simulink model "BatterySOCEstimation"  (R2025b)
settings: Solver=VariableStepAuto  StartTime=0.0  StopTime=6*3600  FixedStep=Ts  RelTol=1e-3  EnableMultiTasking=on
PreLoadFcn:
  | BatterySOCEstimationData;
values from neighbouring files (symbols this model uses):
  R = 0.7    [BatterySOCEstimationData.m]    (also in UTFRBatteryParameters.m = 0.5)
  SOC0 = 0.8    [BatterySOCEstimationData.m]    (also in UTFRBatteryParameters.m = 0.95)
  Ts = 1    [BatterySOCEstimationData.m]    (also in UTFRBatteryParameters.m = 0.01)
libraries: fl_lib x8, nesl_utility x5, simulink x3, batteryecm_lib x1, BatteryEstimators x1
CloseFcn:
  | try
  |     close(h1_BatterySOCEstimation)
  | catch
  | end
  | 
  | clear h1_BatterySOCEstimation
  | 
  | clear BatterySOCEstimationSimlog
  | clear BatterySOCEstimationLogsout
  | 
  | clear AH SOC_vec T_vec R0_mat R1_mat tau1_mat
  | clear V0_mat Q R P0 initialSOC SOC0 Ts
  | clear cell_area h_conv thermal_mass
Description:
  | Battery State-of-Charge Estimation
settings Model: Creator=The MathWorks, Inc.  LastModifiedBy=The MathWorks, Inc.
settings SolverCC: AlgebraicLoopSolver=TrustRegion  AutoInsertRateTranBlk=on  MaxZcPerStep=1.0
settings DataIOCC: MaxDataPoints=370000  ReturnWorkspaceOutputs=off  SignalLoggingName=BatterySOCEstimationLogsout
settings OptimizationCC: ReuseModelBlockBuffer=off  LifeSpan=inf
settings DebuggingCC: UnconnectedInputMsg=warning  UnconnectedOutputMsg=warning  UnconnectedLineMsg=warning  SFUnexpectedBacktrackingDiag=warning  SFNoUnconditionalDefaultTransitionDiag=warning  SFExecutionAtInitializationDiag=none  ArithmeticOperatorsInVariantConditions=warning
settings ModelReferenceCC: EnableRefExpFcnMdlSchedulingChecks=on
settings SFSimCC: SimUseLocalCustomCode=off  CustomCodeUndefinedFunction=UseInterfaceOnly
settings RTWCC: RTWUseLocalCustomCode=off  GPUComputeCapability=3.5  DLArmComputeVersion=19.05
settings CodeAppCC: StateflowObjectComments=on
settings GRTTargetCC: TargetLangStandard=C89/C90 (ANSI)
settings ConfigComp: CovMetricSettings=dw  CovSaveCumulativeToWorkspaceVar=on  CovSaveSingleToWorkspaceVar=on  CovExternalEMLEnable=off
settings SimscapeCC: SimscapeLogType=all  SimscapeLogSimulationStatistics=on  SimscapeLogName=BatterySOCEstimationSimlog  SimscapeLogLimitData=off  SimscapeLogDataHistory=370000.0

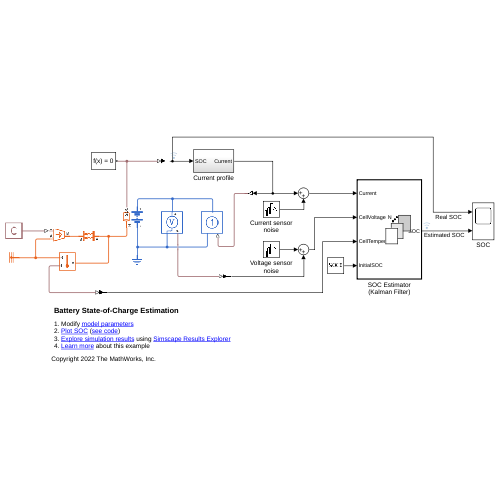
[thumbnail: Simulink's stored preview of the top-level diagram]
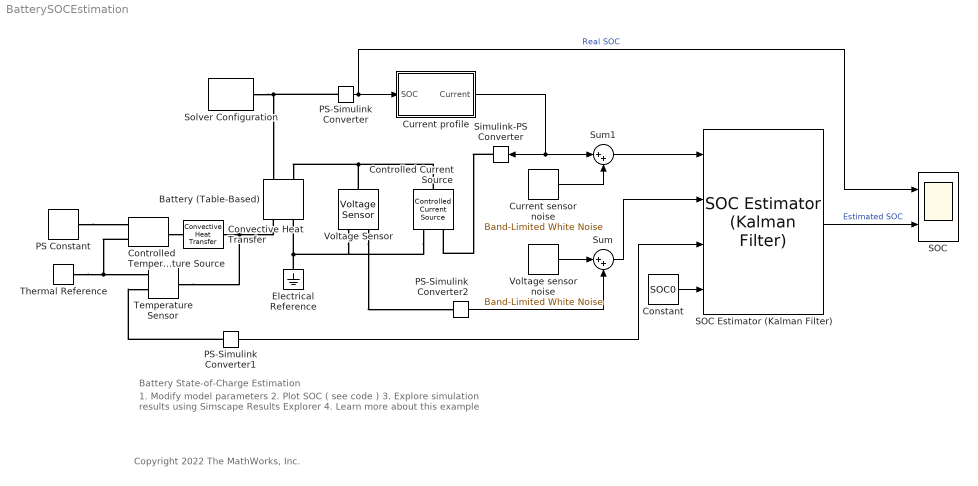
== system BatterySOCEstimation ==
  note: Battery State-of-Charge Estimation
  note: 1. Modify model parameters
      | 2. Plot SOC ( see code )
      | 3. Explore simulation results using Simscape Results Explorer
      | 4. Learn more about this example
  note: Copyright 2022 The MathWorks, Inc.
  Battery (Table-Based) : batteryecm_lib/Battery (Table-Based)  SOC_vec=SOC_vec  T_dependence=simscape.enum.tablebattery.temperature_dependence.yes  prm_dir=simscape.enum.tablebattery.prm_dir.noCurrentDirectionality  T_vec=T_vec K  V0_mat=V0_mat V  V0_vec=[3.5057, 3.566, 3.6337, 3.7127, 3.9259, 4.0777, 4.1928] V  V_range=[0, inf] V  R0_mat=R0_mat Ohm  R0_vec=[.0085, .0085, .0087, .0082, .0083, .0085, .0085] Ohm  R0_dis_mat=[.0117, .0085, .009; .011, .0085, .009; .0114, .0087, .0092; .0107, .0082, .0088; .0107, .0083, .0091; .0113, .0085, .0089; .0116, .0085, .0089] Ohm  R0_dis_vec=[.0085, .0085, .0087, .0082, .0083, .0085, .0085] Ohm  R0_ch_mat=[.0117, .0085, .009; .011, .0085, .009; .0114, .0087, .0092; .0107, .0082, .0088; .0107, .0083, .0091; .0113, .0085, .0089; .0116, .0085, .0089] Ohm  R0_ch_vec=[.0085, .0085, .0087, .0082, .0083, .0085, .0085] Ohm  AH=AH A*hr  prm_leak=simscape.enum.tablebattery.prm_leak.disabled  Rleak_vec=[8000, 7000, 6000] Ohm  Rleak=7e3 Ohm  extrapolation_option=simscape.enum.extrapolation.nearest  SOC_port=simscape.enum.tablebattery.enable.yes  prm_dyn=simscape.enum.tablebattery.prm_dyn.rc1  R1_mat=R1_mat Ohm  R1_vec=[.0029, .0024, .0026, .0016, .0023, .0018, .0017] Ohm  tau1_mat=tau1_mat s  tau1_vec=[36, 45, 105, 29, 77, 33, 39] s  R2_mat=[.0109, .0029, .0013; .0069, .0024, .0012; .0047, .0026, .0013; .0034, .0016, .001; .0033, .0023, .0014; .0033, .0018, .0011; .0028, .0017, .0011] Ohm  R2_vec=[.0029, .0024, .0026, .0016, .0023, .0018, .0017] Ohm  tau2_mat=[20, 36, 39; 31, 45, 39; 109, 105, 61; 36, 29, 26; 59, 77, 67; 40, 33, 29; 25, 39, 33] s  tau2_vec=[36, 45, 105, 29, 77, 33, 39] s  R3_mat=[.0109, .0029, .0013; .0069, .0024, .0012; .0047, .0026, .0013; .0034, .0016, .001; .0033, .0023, .0014; .0033, .0018, .0011; .0028, .0017, .0011] Ohm  R3_vec=[.0029, .0024, .0026, .0016, .0023, .0018, .0017] Ohm  tau3_mat=[20, 36, 39; 31, 45, 39; 109, 105, 61; 36, 29, 26; 59, 77, 67; 40, 33, 29; 25, 39, 33] s  tau3_vec=[36, 45, 105, 29, 77, 33, 39] s  R4_mat=[.0109, .0029, .0013; .0069, .0024, .0012; .0047, .0026, .0013; .0034, .0016, .001; .0033, .0023, .0014; .0033, .0018, .0011; .0028, .0017, .0011] Ohm  R4_vec=[.0029, .0024, .0026, .0016, .0023, .0018, .0017] Ohm  tau4_mat=[20, 36, 39; 31, 45, 39; 109, 105, 61; 36, 29, 26; 59, 77, 67; 40, 33, 29; 25, 39, 33] s  tau4_vec=[36, 45, 105, 29, 77, 33, 39] s  R5_mat=[.0109, .0029, .0013; .0069, .0024, .0012; .0047, .0026, .0013; .0034, .0016, .001; .0033, .0023, .0014; .0033, .0018, .0011; .0028, .0017, .0011] Ohm  R5_vec=[.0029, .0024, .0026, .0016, .0023, .0018, .0017] Ohm  tau5_mat=[20, 36, 39; 31, 45, 39; 109, 105, 61; 36, 29, 26; 59, 77, 67; 40, 33, 29; 25, 39, 33] s  tau5_vec=[36, 45, 105, 29, 77, 33, 39] s  prm_fade=simscape.enum.tablebattery.prm_fade.disabled  N0=10  dV0=0  dR0=500  dAH=0  dRleak=0  dR1=0  dR2=0  dR3=0  dR4=0  dR5=0  N0vec=[100, 200, 300]  Tfadevec=[298.15, 323.15] K  dV0vec=[0, 0, 0]  dR0vec=[0, 0, 0]  dAHvec=[0, 0, 0]  dRleakvec=[0, 0, 0]  dR1vec=[0, 0, 0]  dR2vec=[0, 0, 0]  dR3vec=[0, 0, 0]  dR4vec=[0, 0, 0]  dR5vec=[0, 0, 0]  dV0mat=[0, 0; 0, 0; 0, 0]  dR0mat=[0, 0; 0, 0; 0, 0]  dAHmat=[0, 0; 0, 0; 0, 0]  dRleakmat=[0, 0; 0, 0; 0, 0]  dR1mat=[0, 0; 0, 0; 0, 0]  dR2mat=[0, 0; 0, 0; 0, 0]  dR3mat=[0, 0; 0, 0; 0, 0]  dR4mat=[0, 0; 0, 0; 0, 0]  dR5mat=[0, 0; 0, 0; 0, 0]  prm_age_modeling=simscape.enum.tablebattery.prm_age_modeling.equation  storage_dt_age_vec=[0] d  storage_T_age_vec=[273] K  prm_age_OCV=simscape.enum.tablebattery.prm_age_OCV.OCV  OCV_age=0.9  SOC_age=0.6  prm_age_resistance=simscape.enum.tablebattery.prm_age.disabled  OCV_scaling_age_resistance=2.2134e6  OCV_offset_age_resistance=1.632e6  temp_exp_age_resistance=0.515833569 V  t_exp_age_resistance=0.75  T_age_vec_resistance=[273.15, 298.15, 323.15] K  dt_age_vec_resistance=[90, 180, 270, 360] d  dR0_age_vec=[0, 0, 0]  t_meas_dR0_age=100 d  dR0_age_mat=[0, 0, 0; 0, 0, 0; 0, 0, 0; 0, 0, 0]  prm_age_capacity=simscape.enum.tablebattery.prm_age.disabled  OCV_scaling_age_capacity=1.5097e07  OCV_offset_age_capacity=8.3625e06  temp_exp_age_capacity=0.6011 V  t_exp_age_capacity=0.75  T_age_vec_capacity=[273.15, 298.15, 323.15] K  dt_age_vec_capacity=[90, 180, 270, 360] d  dAH_age_vec=[0, 0, 0]  t_meas_dAH_age=100 d  dAH_age_mat=[0, 0, 0; 0, 0, 0; 0, 0, 0; 0, 0, 0]  thermal_port=simscape.enum.thermaleffects.model  temperature=298.15 K  thermal_mass=thermal_mass J/K  i_specify=off  i_priority=None  i=0 A  i_nominal_specify=off  i_nominal_value=1  i_nominal_unit=A  v_specify=off  v_priority=None  v=0 V  v_nominal_specify=off  v_nominal_value=1  v_nominal_unit=V  stateOfCharge_specify=on  stateOfCharge_priority=High  stateOfCharge=initialSOC  stateOfCharge_nominal_specify=off  stateOfCharge_nominal_value=1  stateOfCharge_nominal_unit=1  num_cycles_specify=off  num_cycles_priority=High  num_cycles=0  num_cycles_nominal_specify=off  num_cycles_nominal_value=1  num_cycles_nominal_unit=1  cell_temperature_specify=off  cell_temperature_priority=High  cell_temperature=293.15 K  cell_temperature_nominal_specify=off  cell_temperature_nominal_value=1  cell_temperature_nominal_unit=K
  Constant : Constant  Value=SOC0
  Controlled Temperature Source : fl_lib/Thermal/Thermal Sources/Controlled Temperature Source
  Controlled Current Source : fl_lib/Electrical/Electrical Sources/Controlled Current Source
  Convective Heat Transfer : fl_lib/Thermal/Thermal Elements/Convective Heat Transfer  thermal_type=foundation.enum.constant_variable.constant  area=cell_area m^2  heat_tr_coeff=h_conv W/(K*m^2)  min_heat_tr_coeff=1e-3 W/(K*m^2)  T_specify=off  T_priority=None  T=0 K  T_nominal_specify=off  T_nominal_value=1  T_nominal_unit=K  Q_specify=off  Q_priority=None  Q=0 W  Q_nominal_specify=off  Q_nominal_value=1  Q_nominal_unit=W
  Current profile : Subsystem
  Current sensor noise : simulink/Sources/Band-Limited White Noise  Cov=1e-2  Ts=1  seed=1234
  Electrical Reference : fl_lib/Electrical/Electrical Elements/Electrical Reference
  PS Constant : fl_lib/Physical Signals/Sources/PS Constant  constant=292.15 K
  PS-Simulink Converter : nesl_utility/PS-Simulink Converter  PhysicalDomain=network_engine_domain  SubClassName=ps_output  LeftPortType=input  RightPortType=output  PseudoPeriodic=off  Frequencies=[]  VectorFormat=inherit  Unit=inherit  AffineConversion=off
  PS-Simulink Converter1 : nesl_utility/PS-Simulink Converter  PhysicalDomain=network_engine_domain  SubClassName=ps_output  LeftPortType=input  RightPortType=output  PseudoPeriodic=off  Frequencies=[]  VectorFormat=inherit  Unit=inherit  AffineConversion=off
  PS-Simulink Converter2 : nesl_utility/PS-Simulink Converter  PhysicalDomain=network_engine_domain  SubClassName=ps_output  LeftPortType=input  RightPortType=output  PseudoPeriodic=off  Frequencies=[]  VectorFormat=inherit  Unit=inherit  AffineConversion=off
  SOC : Scope  NumInputPorts=2
      settings: ActiveDisplayYMinimum=0.20845  ActiveDisplayYMaximum=0.98731  DataLoggingVariableName=ScopeData3
  SOC Estimator (Kalman Filter) : BatteryEstimators/SOC Estimator (Kalman Filter)  CurrentInputPartition=off  filterType=Extended Kalman filter  alpha=1  beta=2  kappa=0  Q=Q  Q_2RC=|  R=R  P0=P0  P0_2RC=[1e-5 0 0; 0 1 0;0 0 1]  Ts=Ts  chargeDynamics=One time-constant dynamics  SOC_vec=SOC_vec  T_vec=T_vec  R0_mat=R0_mat  R1_mat=R1_mat  tau1_mat=tau1_mat  R2_mat=[.0109, .0029, .0013; .0069, .0024, .0012; .0047, .0026, .0013; .0034, .0016, .001; .0033, .0023, .0014; .0033, .0018, .0011; .0028, .0017, .0011]  tau2_mat=[20, 36, 39; 31, 45, 39; 109, 105, 61; 36, 29, 26; 59, 77, 67; 40, 33, 29; 25, 39, 33]  V0_mat=V0_mat  AH=AH  DataType=Inherit: auto
      | [1e-6 0 0;
      | 0 1e-6 0; 0 0 1e-6]
  Simulink-PS Converter : nesl_utility/Simulink-PS Converter  PhysicalDomain=network_engine_domain  SubClassName=ps_input  LeftPortType=input  RightPortType=output  PseudoPeriodic=off  Frequencies=[]  NoiseDistribution=none  NoiseParameters=[]  Unit=1  AffineConversion=off  FilteringAndDerivatives=provide  SimscapeFilterOrder=1  InputFilterTimeConstant=0.001  UdotUserProvided=0
  Solver Configuration : nesl_utility/Solver Configuration  PhysicalDomain=network_engine_domain  SubClassName=solver  LeftPortType=input  RightPortType=generic  Tones=[]  Harmonics=[]  SimulateNoise=off  Profile=off  UseLocalSampling=off  EnableSwitchedLinearOptims=on  FrequencyDomain=off  UseCCode=off  RelTol=0.001  AbsTol=0.001  MinStep=1e-09  ToWorkspace=off  RevertToSquareIcSolve=off  NumHomotopyIterations=100  PhasorMode=off  PhasorModeNumHarmonics=1  ConsistencySolver=NEWTON_XTOL_AFTER_FTOL  IndexReductionMethod=DerivativeReplacement  DoDC=off  ResidualTolerance=1e-09  ConsistencyTolSource=GLOBAL  ConsistencyAbsTol=0.001  ConsistencyRelTol=0.001  ConsistencyTolFactor=0.001  UseLocalSolver=on  LocalSolverChoice=NE_BACKWARD_EULER_ADVANCER  ResolveIndetEquations=on  FunctionEvalNumThread=1  LocalSolverSampleTime=1  DoFixedCost=on  MaxNonlinIter=3  MaxModeIter=2  ComputeImpulses=off  ImpulseIterations=2  LinearAlgebra=auto  LinearAlgebraNumThread=0  EquationFormulation=NE_TIME_EF  DelaysMemoryBudget=1024  AutomaticFiltering=on  FilteringTimeConstant=0.001  PartitionStorageMethod=AS_NEEDED  PartitionMemoryBudget=1024  PartitionMethod=ROBUST  MultibodyUseLocalSolver=off  MultibodyLocalSolverChoice=ODE1  MultibodyLocalSolverSampleTime=0.001
  Sum : Sum  Inputs=|++
  Sum1 : Sum  Inputs=|++
  Temperature Sensor : fl_lib/Thermal/Thermal Sensors/Temperature Sensor  temperature_measure=foundation.enum.MeasurementReference.difference
  Thermal Reference : fl_lib/Thermal/Thermal Elements/Thermal Reference
  Voltage Sensor : fl_lib/Electrical/Electrical Sensors/Voltage Sensor
  Voltage sensor noise : simulink/Sources/Band-Limited White Noise  Cov=1e-2  Ts=1  seed=1234
  wires:
  PS-Simulink Converter2/1 -> Sum/2
  Current sensor noise/1 -> Sum1/2
  Sum1/1 -> SOC Estimator (Kalman Filter)/1
  Sum/1 -> SOC Estimator (Kalman Filter)/2
  PS-Simulink Converter1/1 -> SOC Estimator (Kalman Filter)/3
  Constant/1 -> SOC Estimator (Kalman Filter)/4
  SOC Estimator (Kalman Filter)/1 -> SOC/2  "Estimated SOC"
  PS-Simulink Converter/1 -> SOC/1, Current profile/1(SOC)  "Real SOC"
  Voltage sensor noise/1 -> Sum/1
  Current profile/1(Current) -> Sum1/1, Simulink-PS Converter/1
  connections:
  PS-Simulink Converter/LConn1 -- Solver Configuration/RConn1 -- Battery (Table-Based)/LConn2
  Convective Heat Transfer/LConn1 -- Temperature Sensor/LConn1 -- Battery (Table-Based)/RConn2
  Controlled Temperature Source/LConn1 -- Convective Heat Transfer/RConn1
  Thermal Reference/LConn1 -- Controlled Temperature Source/RConn2 -- Temperature Sensor/RConn1
  PS-Simulink Converter1/LConn1 -- Temperature Sensor/RConn2
  Electrical Reference/LConn1 -- Voltage Sensor/RConn2 -- Controlled Current Source/RConn2 -- Battery (Table-Based)/RConn1
  Voltage Sensor/LConn1 -- Controlled Current Source/LConn1 -- Battery (Table-Based)/LConn1
  Simulink-PS Converter/RConn1 -- Controlled Current Source/RConn1
  Voltage Sensor/RConn1 -- PS-Simulink Converter2/LConn1
  PS Constant/RConn1 -- Controlled Temperature Source/RConn1

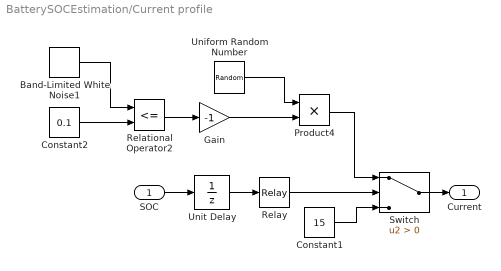
== system BatterySOCEstimation/Current profile ==
  SOC : Inport
  Band-Limited White Noise1 : simulink/Sources/Band-Limited White Noise  Cov=1  Ts=50  seed=[23341]
  Constant1 : Constant  Value=15
  Constant2 : Constant  Value=0.1
  Gain : Gain  Gain=-1
  Product4 : Product
  Relational Operator2 : RelationalOperator  Operator=<=  OutDataTypeStr=boolean  RndMeth=Simplest  InputSameDT=off
  Relay : Relay  OnSwitchValue=0.9  OffSwitchValue=0.3  OffOutputValue=-1
  Switch : Switch  Criteria=u2 > Threshold  SaturateOnIntegerOverflow=off  InputSameDT=off
  Uniform Random Number : UniformRandomNumber  Minimum=5  Maximum=55  SampleTime=100
  Unit Delay : UnitDelay  SampleTime=Ts  HasFrameUpgradeWarning=on
  Current : Outport
  wires:
  SOC/1 -> Unit Delay/1
  Constant1/1 -> Switch/3
  Relay/1 -> Switch/2
  Product4/1 -> Switch/1
  Unit Delay/1 -> Relay/1
  Switch/1 -> Current/1
  Uniform Random Number/1 -> Product4/1
  Band-Limited White Noise1/1 -> Relational Operator2/1
  Gain/1 -> Product4/2
  Relational Operator2/1 -> Gain/1
  Constant2/1 -> Relational Operator2/2
